simulink model "MidPoint_Bridge_Cycloconverter_R_Load"  (R2023b)
settings: Solver=VariableStepAuto  StartTime=0.0  StopTime=1  RelTol=1e-3
libraries: spsMosfetLib x4, spsACVoltageSourceLib x2, spsVoltageMeasurementLib x2, spsSeriesRLCBranchLib x1, sps_lib x1
settings Model: Creator=Anuj  LastModifiedBy=Anuj

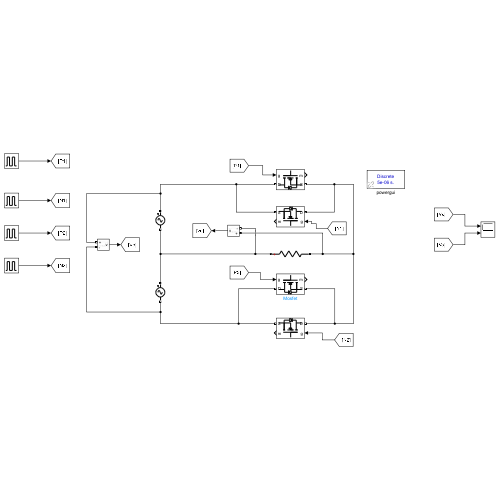
[thumbnail: Simulink's stored preview of the top-level diagram]
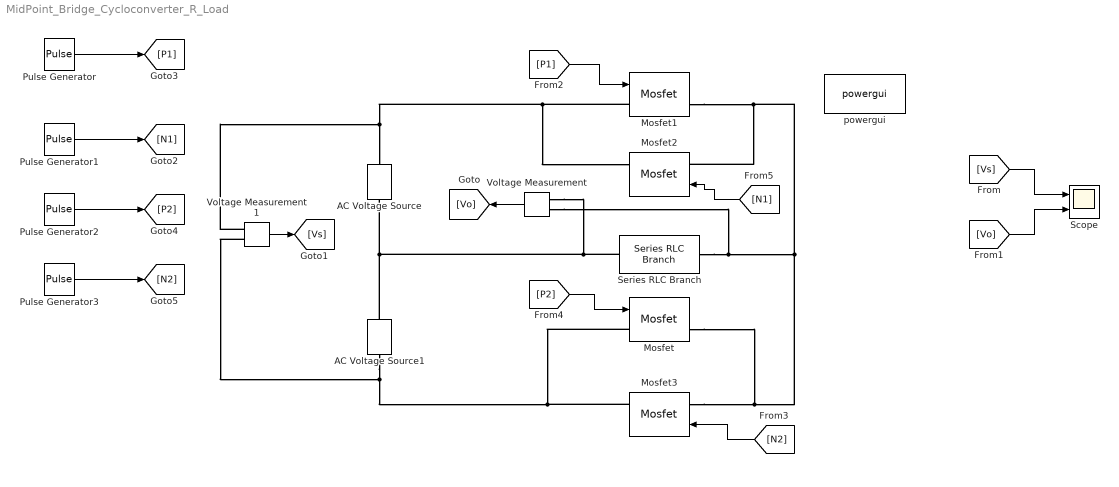
== system MidPoint_Bridge_Cycloconverter_R_Load ==
  AC Voltage Source : spsACVoltageSourceLib/AC Voltage Source  Amplitude=30*sqrt(2)  Phase=0  Frequency=50  SampleTime=0  Measurements=None  BusType=swing  Pref=10e3  Qref=0  Qmin=-inf  Qmax=+inf
  AC Voltage Source1 : spsACVoltageSourceLib/AC Voltage Source  Amplitude=30*sqrt(2)  Phase=0  Frequency=50  SampleTime=0  Measurements=None  BusType=swing  Pref=10e3  Qref=0  Qmin=-inf  Qmax=+inf
  Mosfet{,1..3} (4 alike) : spsMosfetLib/Mosfet  Ron=0.1  Lon=0  Rd=0.01  Vfd=0  IC=0  Rs=1e5  Cs=inf  Measurements=on
  Pulse Generator : DiscretePulseGenerator  PulseType=Time based  Period=0.02  PulseWidth=25  PhaseDelay=(0.02)*(30/360)
  Pulse Generator1 : DiscretePulseGenerator  PulseType=Time based  Period=0.002  PulseWidth=25  PhaseDelay=0.002*((360+30)/360)
  Pulse Generator2 : DiscretePulseGenerator  PulseType=Time based  Period=0.002  PulseWidth=25  PhaseDelay=0.002*((180+30)/360)
  Pulse Generator3 : DiscretePulseGenerator  PulseType=Time based  Period=0.002  PulseWidth=25  PhaseDelay=0.002*((540+30)/360)
  Scope : Scope  NumInputPorts=2
  Series RLC Branch : spsSeriesRLCBranchLib/Series RLC Branch  LConnTagsString=__new0  RConnTagsString=__new0  BranchType=R  Resistance=10  Inductance=1e-3  SetiL0=off  InitialCurrent=0  Capacitance=1e-6  Setx0=off  InitialVoltage=0  Measurements=None
  Voltage Measurement : spsVoltageMeasurementLib/Voltage Measurement  PhasorSimulation=off  OutputType=Complex  PSBequivalent=0
  Voltage Measurement1 : spsVoltageMeasurementLib/Voltage Measurement  PhasorSimulation=off  OutputType=Complex  PSBequivalent=0
  powergui : sps_lib/powergui  Priority=1  SimulationMode=Discrete  SampleTime=5e-6  frequency=60  Iterations=50  frequencyindice=50  Pbase=100e6  ErrMax=1e-4  UnitsV=kV  UnitsW=MW  buscounter=0  FunctionMessages=off  echomessages=off  EnableUseOfTLC=off  CurrentSourceSwitches=off  DisableSnubberDevices=off  DisableRonSwitches=off  DisableVfSwitches=off  DisplayEquations=off  AutomaticDiscreteSolvers=off  SolverType=Tustin/Backward Euler (TBE)  Interpol=off  ExternalGateDelay=off  methode=off  Ts=100  x0status=blocks  SPID=on  SwTol=0  HookPort=off  NonlinearTolerance=1e-4  nMaxIteration=100  ContinueOnMaxIteration=off  RestoreLinks=warning  ResistiveCurrentMeasurement=off  Frange=[0:2:500]  Ylog=off  Xlog=on  ShowGrid=off  save=off  variable=ZData  structure=0  ZoomFFT=off  StartTime=0.0  cycles=1  DisplayStyle=1  fundamental=60  FreqAxis=off  MaxFrequency=1000  frequencyindicesteady=1  RmsSteady=1  display=off
  wires:
  Voltage Measurement/1 -> [Vo]
  Voltage Measurement1/1 -> [Vs]
  [Vs] -> Scope/1
  [Vo] -> Scope/2
  [P1] -> Mosfet1/1
  [N2] -> Mosfet3/1
  [P2] -> Mosfet/1
  [N1] -> Mosfet2/1
  Pulse Generator/1 -> [P1]
  Pulse Generator1/1 -> [N1]
  Pulse Generator2/1 -> [P2]
  Pulse Generator3/1 -> [N2]
  connections:
  Mosfet2/RConn1 -- Mosfet1/LConn1 -- AC Voltage Source/RConn1 -- Voltage Measurement1/LConn1
  AC Voltage Source1/RConn1 -- Voltage Measurement/LConn2 -- Series RLC Branch/LConn1 -- AC Voltage Source/LConn1
  Mosfet3/LConn1 -- Mosfet/RConn1 -- Voltage Measurement/LConn1 -- Series RLC Branch/RConn1 -- Mosfet2/LConn1 -- Mosfet1/RConn1
  AC Voltage Source1/LConn1 -- Voltage Measurement1/LConn2 -- Mosfet3/RConn1 -- Mosfet/LConn1
